simulink library "DCT_Vehicle_Dynamics_Lib"  (R2025a)
settings: Solver=ode45  StartTime=0.0  StopTime=10.0  RelTol=1e-3  EnableMultiTasking=on
undefined symbols (not defined in the file): DCT_Param
libraries: fl_lib x26, nesl_utility x9, sdl_lib x5
Description:
  | Copyright 2014-2025 The MathWorks, Inc.
settings Model: Creator=smiller  LastModifiedBy=smiller
settings SolverCC: AlgebraicLoopSolver=TrustRegion
settings DataIOCC: LimitDataPoints=on  SaveFormat=Array  SignalLoggingSaveFormat=ModelDataLogs  ReturnWorkspaceOutputs=off
settings OptimizationCC: ReuseModelBlockBuffer=off  ExpressionDepthLimit=2147483647.0  LifeSpan=inf
settings DebuggingCC: UnderspecifiedInitializationDetection=Classic  MergeDetectMultiDrivingBlocksExec=none  SolverPrmCheckMsg=warning  FcnCallInpInsideContextMsg=warning  UnconnectedInputMsg=warning  UnconnectedOutputMsg=warning  UnconnectedLineMsg=warning  AllowSymbolicDim=off  StateNameClashWarn=warning  PregeneratedLibrarySubsystemCodeDiagnostic=none  SFUnexpectedBacktrackingDiag=warning  SFNoUnconditionalDefaultTransitionDiag=warning  SFExecutionAtInitializationDiag=none  ArithmeticOperatorsInVariantConditions=warning
settings HardwareCC: ProdBitPerPointer=32.0  ProdBitPerSizeT=32.0  ProdBitPerPtrDiffT=32.0  ProdLargestAtomicFloat=None  ProdIntDivRoundTo=Undefined  ProdEndianess=Unspecified  ProdWordSize=32.0  ProdHWDeviceType=32-bit Generic
settings ModelReferenceCC: EnableRefExpFcnMdlSchedulingChecks=on  PropagateSignalLabelsOutOfModel=off
settings SFSimCC: SimUseLocalCustomCode=off  CustomCodeUndefinedFunction=UseInterfaceOnly
settings RTWCC: RTWUseLocalCustomCode=off  GPUComputeCapability=3.5  DLArmComputeVersion=19.05
settings CodeAppCC: StateflowObjectComments=on
settings GRTTargetCC: TargetLangStandard=C89/C90 (ANSI)  CombineOutputUpdateFcns=off  GRTInterface=on
settings ConfigComp: CovMetricSettings=dw  CovSaveCumulativeToWorkspaceVar=on  CovSaveSingleToWorkspaceVar=on  CovExternalEMLEnable=off  CovSFcnEnable=off

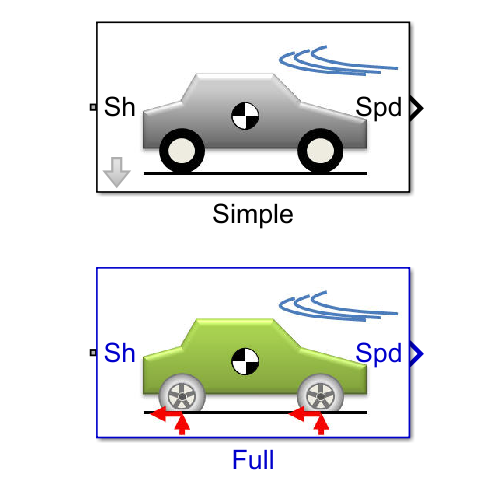
[thumbnail: Simulink's stored preview of the top-level diagram]
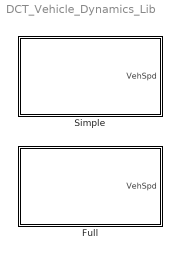
== system DCT_Vehicle_Dynamics_Lib ==
  Full : Subsystem
      mask Display:
      | image(imread('DCT_Vehicle_Dynamics_Full_IMAGE.jpg'));
      | port_label('LConn',1,'Sh');
      | port_label('output',1,'Spd');
  Simple : Subsystem  mask(Rigid vehicle model){mass=DCT_Param.Vehicle.Mass, area=DCT_Param.Vehicle.Frontal_Area, Cd=DCT_Param.Vehicle.Aero_Drag_Coeff, radius=DCT_Param.Vehicle.Tire.Radius, wheel_inertia=DCT_Param.Vehicle.Tire.Inertia, gear_ratio=DCT_Param.Vehicle.Final_Drive_Ratio}
      mask prompts: mass "Vehicle mass (Kg)"; area "Vehicle Area (m^2)"; Cd "Aerodynamic drag coefficient (unitless)"; radius "Tire radius (m)"; wheel_inertia "Total wheel inertia (kg*m^2)"; gear_ratio "Engine to vehicle gear ratio"
      mask help: Model vehicle effective inertia and drag force as seen by the engine. It is assumed that the vehicle is moving on flat terrain. No bearing friction or gear losses are included.
      mask init:
      | gravity = 9.81;
      mask Display:
      | image(imread('DCT_Vehicle_Dynamics_Simple_IMAGE.jpg'));
      | port_label('LConn',1,'Sh');
      | port_label('output',1,'Spd');

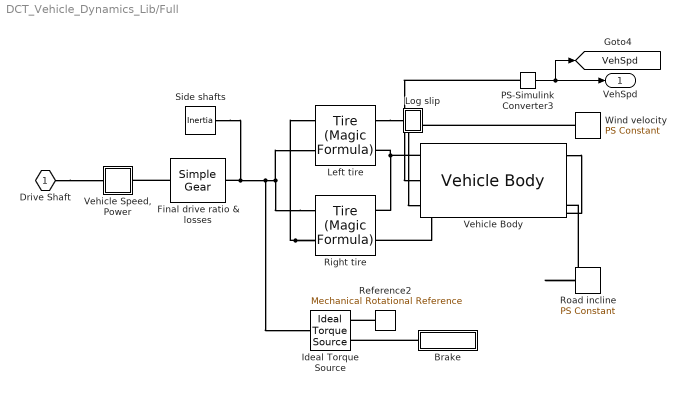
== system DCT_Vehicle_Dynamics_Lib/Full ==
  Brake : Subsystem
  Final drive ratio & losses : sdl_lib/Gears/Simple Gear  ratio=DCT_Param.Vehicle.Final_Drive_Ratio  rotation_direction=3-2*(2)  friction_model=1  T_noload=0.1 N*m  T_nom=5 N*m  efficiency_nom=0.8  efficiency=DCT_Param.Vehicle.Final_Drive_Efficiency  temperature_TLU=[ 280 300 320 ] K  load_TLU=[ 1 5 10 ] N*m  efficiency_TLU=[ 0.95 0.9 0.85 ]  efficiency_TLU2=[ 0.85 0.8 0.75; 0.95 0.9 0.85; 0.85 0.8 0.7 ]  w_thr=DCT_Param.Vehicle.Final_Drive_Vel_Thresh rad/s  pwr_thr=0.001 W  enable_backlash=false  hardstop_model=simscape.enum.hardstop.smooth  backlash_distance=1e-3 mm  r_base=0.1 m  transition=1e-4 mm  backlash_stiffness=1e7 N/m  backlash_damping=1e6 N*s/m  coeff_rest=0  v_tol=0.001 m/s  f_tol=0 N  mu_visc=[0 0] N*m/(rad/s)  thermal_mass=50 J/K  temperature_specify=off  temperature_priority=High  temperature=300 K  temperature_nominal_specify=off  temperature_nominal_value=1  temperature_nominal_unit=K  x_backlash_specify=off  x_backlash_priority=None  x_backlash=0 mm  x_backlash_nominal_specify=off  x_backlash_nominal_value=1  x_backlash_nominal_unit=mm  f_hardstop_specify=off  f_hardstop_priority=None  f_hardstop=0 N  f_hardstop_nominal_specify=off  f_hardstop_nominal_value=1  f_hardstop_nominal_unit=N  v_backlash_specify=off  v_backlash_priority=None  v_backlash=0 m/s  v_backlash_nominal_specify=off  v_backlash_nominal_value=1  v_backlash_nominal_unit=m/s
  Ideal Torque Source : fl_lib/Mechanical/Mechanical Sources/Ideal Torque Source
  Left tire : sdl_lib/Tires & Vehicles/Tire (Magic Formula)  parameterization=3  F_z1=3000 N  F_x1=3500 N  kappa1=10  B_m=10  C_m=1.9  D_m=1  E_m=0.97  fz0=DCT_Param.Vehicle.Tire.Nominal_Vertical_Load N  p_Cx=DCT_Param.Vehicle.Tire.C_Coeff  p_Dx=DCT_Param.Vehicle.Tire.D_Coeff  p_Ex=DCT_Param.Vehicle.Tire.E_Coeff  p_Kx=DCT_Param.Vehicle.Tire.BCD_Coeff  p_Hx=DCT_Param.Vehicle.Tire.H_Coeff  p_Vx=DCT_Param.Vehicle.Tire.V_Coeff  rolling_radius_model=sdl.enum.RollingRadiusParameterization.Constant  r_e=DCT_Param.Vehicle.Tire.Radius m  r_0=0.3 m  breff=8.39  dreff=0.26  freff=0.074  q_re0=0.99  q_v1=0.008  longvl=17 m/s  cz=5e5 N/m  model_resistance=0  resistance_model=1  coeff=0.015  p_tire=250e3 Pa  alpha=-0.003  beta=0.97  coeff_a=84e-4  coeff_b=6.2e-4 s/m  coeff_c=1.6e-4 s^2/m^2  p_tire0=240e3 Pa  fz0_resistance=4000 N  vH0=16 m/s  q_Sy=[.0082, 0, .0014, .001, 0, 0, 1.08, -.5]  v_thr=1e-3 m/s  enable_scaling_coefficients=false  lfzO=1  lcx=1  lmux=1  lex=1  lkx=1  lhx=1  lvx=1  lmy=1  model_compliance=0  stiffness=1e+6 N/m  damping=1000 N/(m/s)  model_inertia=1  inertia=DCT_Param.Vehicle.Tire.Inertia kg*m^2  initial_velocity=DCT_Param.Vehicle.Tire.Initial_Velocity rpm  vxlow=DCT_Param.Vehicle.Tire.Slip_Vel_Thresh m/s  v_tr_thr=0.1*(DCT_Param.Vehicle.Tire.Slip_Vel_Thresh) m/s  kpumin=-1e5  kpumax=1e5
  Log slip : Subsystem
  PS-Simulink Converter3 : nesl_utility/PS-Simulink Converter  PhysicalDomain=network_engine_domain  SubClassName=ps_output  LeftPortType=input  RightPortType=output  PseudoPeriodic=off  Frequencies=[]  VectorFormat=1-D array  Unit=km/hr  AffineConversion=off
  Reference2 : fl_lib/Mechanical/Rotational Elements/Mechanical Rotational Reference
  Right tire : sdl_lib/Tires & Vehicles/Tire (Magic Formula)  parameterization=3  F_z1=3000 N  F_x1=3500 N  kappa1=10  B_m=10  C_m=1.9  D_m=1  E_m=0.97  fz0=DCT_Param.Vehicle.Tire.Nominal_Vertical_Load N  p_Cx=DCT_Param.Vehicle.Tire.C_Coeff  p_Dx=DCT_Param.Vehicle.Tire.D_Coeff  p_Ex=DCT_Param.Vehicle.Tire.E_Coeff  p_Kx=DCT_Param.Vehicle.Tire.BCD_Coeff  p_Hx=DCT_Param.Vehicle.Tire.H_Coeff  p_Vx=DCT_Param.Vehicle.Tire.V_Coeff  rolling_radius_model=sdl.enum.RollingRadiusParameterization.Constant  r_e=DCT_Param.Vehicle.Tire.Radius m  r_0=0.3 m  breff=8.39  dreff=0.26  freff=0.074  q_re0=0.99  q_v1=0.008  longvl=17 m/s  cz=5e5 N/m  model_resistance=0  resistance_model=1  coeff=0.015  p_tire=250e3 Pa  alpha=-0.003  beta=0.97  coeff_a=84e-4  coeff_b=6.2e-4 s/m  coeff_c=1.6e-4 s^2/m^2  p_tire0=240e3 Pa  fz0_resistance=4000 N  vH0=16 m/s  q_Sy=[.0082, 0, .0014, .001, 0, 0, 1.08, -.5]  v_thr=1e-3 m/s  enable_scaling_coefficients=false  lfzO=1  lcx=1  lmux=1  lex=1  lkx=1  lhx=1  lvx=1  lmy=1  model_compliance=0  stiffness=1e+6 N/m  damping=1000 N/(m/s)  model_inertia=1  inertia=DCT_Param.Vehicle.Tire.Inertia kg*m^2  initial_velocity=DCT_Param.Vehicle.Tire.Initial_Velocity rpm  vxlow=DCT_Param.Vehicle.Tire.Slip_Vel_Thresh m/s  v_tr_thr=0.1*(DCT_Param.Vehicle.Tire.Slip_Vel_Thresh) m/s  kpumin=-1e5  kpumax=1e5
  Road incline : fl_lib/Physical Signals/Sources/PS Constant  constant=0
  Side shafts : fl_lib/Mechanical/Rotational Elements/Inertia  inertia=DCT_Param.Vehicle.Side_Shaft_Inertia kg*m^2  num_ports=foundation.enum.numPorts2.one  w_specify=on  w_priority=High  w=DCT_Param.Vehicle.Side_Shaft_Initial_Velocity rad/s  w_nominal_specify=off  w_nominal_value=1  w_nominal_unit=rad/s  t_specify=off  t_priority=High  t=0 N*m  t_nominal_specify=off  t_nominal_value=1  t_nominal_unit=N*m
  Vehicle Body : sdl_lib/Tires & Vehicles/Vehicle Body  mass=DCT_Param.Vehicle.Mass kg  n_w=DCT_Param.Vehicle.Wheels_Per_Axle  x_f=DCT_Param.Vehicle.Distance_CG_FrontAxle m  x_r=DCT_Param.Vehicle.Distance_CG_RearAxle m  y_c=DCT_Param.Vehicle.Distance_CG_Ground m  mass_var=simscape.enum.onoff.off  g=9.81 m/s^2  liftoff_warning=simscape.enum.onoff.off  area=DCT_Param.Vehicle.Frontal_Area m^2  Cd_var=false  Cd=DCT_Param.Vehicle.Aero_Drag_Coeff  rho=1.18 kg/m^3  model_pitch=simscape.enum.onoff.off  inertia=4000 kg*m^2  suspension_model=sdl.enum.linearTLU.linear  k_f=1e4 N/m  b_f=1e4 N/(m/s)  k_r=1e4 N/m  b_r=1e4 N/(m/s)  k_f_TLU=[-2000, -1000, 0, 1000, 2000] N  x_f_TLU=[-.4, -.2, 0, .2, .4] m  b_f_TLU=[-200, -100, 0, 100, 200] N  v_f_TLU=[-4, -2, 0, 2, 4] m/s  k_r_TLU=[-2000, -1000, 0, 1000, 2000] N  x_r_TLU=[-.4, -.2, 0, .2, .4] m  b_r_TLU=[-200, -100, 0, 100, 200] N  v_r_TLU=[-4, -2, 0, 2, 4] m/s  interp_method=simscape.enum.interpolation.linear  extrap_method=simscape.enum.extrapolation.linear  model_hardstop=simscape.enum.onoff.off  upper_bound_f=.25 m  lower_bound_f=-.25 m  stop_k_f=1e6 N/m  stop_b_f=150 N/(m/s)  upper_bound_r=.25 m  lower_bound_r=-.25 m  stop_k_r=1e6 N/m  stop_b_r=150 N/(m/s)  initial_pitch=0 rad  initial_pitch_rate=0 rad/s  v_specify=on  v_priority=High  v=DCT_Param.Vehicle.Initial_Velocity m/s  v_nominal_specify=off  v_nominal_value=1  v_nominal_unit=m/s
      settings: InternalSimscapePortConfiguration="{\"Bottom\":[{\"id\":\"NR\",\"label\":\"NR\",\"type\":\"output\"},{\"id\":\"NF\",\"label\":\"NF\",\"type\":\"output\"},{\"id\":\"beta\",\"label\":\"beta\",\"type\":\"input\"}],\"Left\":[{\"id\":\"H\",\"label\":\"H\",\"type\":\"foundation.mechanical.translational.translational\"}],\"Right\":[],\"Top\":[{\"id\":\"V\",\"label\":\"V\",\"type\":\"output\"},{\"id\":\"wind\",\"label\":\"W\",\"type\":\"input\"}]}"
  "Vehicle Speed, Power" : Subsystem
      mask Display: disp('S')
  Wind velocity : fl_lib/Physical Signals/Sources/PS Constant  constant=0
  Drive Shaft : PMIOPort  Side=Left
  VehSpd : Outport  VectorParamsAs1DForOutWhenUnconnected=off
  tag scope: VehSpd=global
  wires:
  PS-Simulink Converter3/1 -> VehSpd/1, [VehSpd]
  connections:
  Vehicle Body/LConn1 -- Right tire/RConn2 -- Left tire/RConn2
  Right tire/LConn1 -- Left tire/LConn1 -- Vehicle Body/RConn1
  Road incline/RConn1 -- Vehicle Body/RConn3
  Wind velocity/RConn1 -- Vehicle Body/LConn3
  PS-Simulink Converter3/LConn1 -- Vehicle Body/LConn2
  Left tire/RConn1 -- Log slip/LConn1
  Drive Shaft/RConn1 -- "Vehicle Speed, Power"/LConn1
  Brake/RConn1 -- Ideal Torque Source/RConn1
  Reference2/LConn1 -- Ideal Torque Source/RConn2
  Final drive ratio & losses/LConn1 -- "Vehicle Speed, Power"/RConn1
  Right tire/LConn2 -- Left tire/LConn2 -- Final drive ratio & losses/RConn1 -- Side shafts/LConn1 -- Ideal Torque Source/LConn1

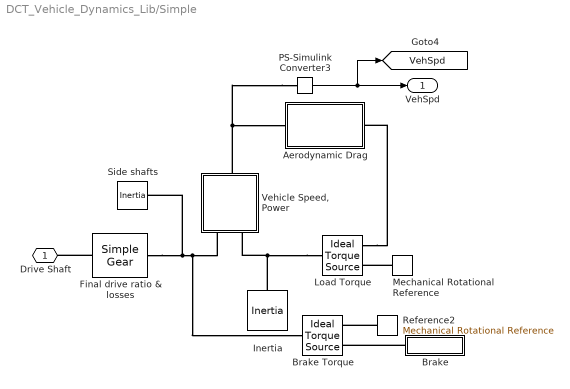
== system DCT_Vehicle_Dynamics_Lib/Simple ==
  Aerodynamic Drag : Subsystem
  Brake : Subsystem
  Brake Torque : fl_lib/Mechanical/Mechanical Sources/Ideal Torque Source
  Final drive ratio & losses : sdl_lib/Gears/Simple Gear  ratio=gear_ratio  rotation_direction=3-2*(2)  friction_model=1  T_noload=0.1 N*m  T_nom=5 N*m  efficiency_nom=0.8  efficiency=DCT_Param.Vehicle.Final_Drive_Efficiency  temperature_TLU=[ 280 300 320 ] K  load_TLU=[ 1 5 10 ] N*m  efficiency_TLU=[ 0.95 0.9 0.85 ]  efficiency_TLU2=[ 0.85 0.8 0.75; 0.95 0.9 0.85; 0.85 0.8 0.7 ]  w_thr=DCT_Param.Vehicle.Final_Drive_Vel_Thresh rad/s  pwr_thr=0.001 W  enable_backlash=false  hardstop_model=simscape.enum.hardstop.smooth  backlash_distance=1e-3 mm  r_base=0.1 m  transition=1e-4 mm  backlash_stiffness=1e7 N/m  backlash_damping=1e6 N*s/m  coeff_rest=0  v_tol=0.001 m/s  f_tol=0 N  mu_visc=[0 0] N*m/(rad/s)  thermal_mass=50 J/K  temperature_specify=off  temperature_priority=High  temperature=300 K  temperature_nominal_specify=off  temperature_nominal_value=1  temperature_nominal_unit=K  x_backlash_specify=off  x_backlash_priority=None  x_backlash=0 mm  x_backlash_nominal_specify=off  x_backlash_nominal_value=1  x_backlash_nominal_unit=mm  f_hardstop_specify=off  f_hardstop_priority=None  f_hardstop=0 N  f_hardstop_nominal_specify=off  f_hardstop_nominal_value=1  f_hardstop_nominal_unit=N  v_backlash_specify=off  v_backlash_priority=None  v_backlash=0 m/s  v_backlash_nominal_specify=off  v_backlash_nominal_value=1  v_backlash_nominal_unit=m/s
  Inertia : fl_lib/Mechanical/Rotational Elements/Inertia  inertia=mass*radius*radius kg*m^2  num_ports=foundation.enum.numPorts2.one  w_specify=on  w_priority=High  w=0 rad/s  w_nominal_specify=off  w_nominal_value=1  w_nominal_unit=rad/s  t_specify=off  t_priority=High  t=0 N*m  t_nominal_specify=off  t_nominal_value=1  t_nominal_unit=N*m
  Load Torque : fl_lib/Mechanical/Mechanical Sources/Ideal Torque Source
  Mechanical Rotational Reference : fl_lib/Mechanical/Rotational Elements/Mechanical Rotational Reference
  PS-Simulink Converter3 : nesl_utility/PS-Simulink Converter  PhysicalDomain=network_engine_domain  SubClassName=ps_output  LeftPortType=input  RightPortType=output  PseudoPeriodic=off  Frequencies=[]  VectorFormat=1-D array  Unit=km/hr  AffineConversion=off
  Reference2 : fl_lib/Mechanical/Rotational Elements/Mechanical Rotational Reference
  Side shafts : fl_lib/Mechanical/Rotational Elements/Inertia  inertia=DCT_Param.Vehicle.Side_Shaft_Inertia+2*wheel_inertia kg*m^2  num_ports=foundation.enum.numPorts2.one  w_specify=on  w_priority=High  w=DCT_Param.Vehicle.Side_Shaft_Initial_Velocity rad/s  w_nominal_specify=off  w_nominal_value=1  w_nominal_unit=rad/s  t_specify=off  t_priority=High  t=0 N*m  t_nominal_specify=off  t_nominal_value=1  t_nominal_unit=N*m
  "Vehicle Speed, Power" : Subsystem
  Drive Shaft : PMIOPort  Side=Left
  VehSpd : Outport  VectorParamsAs1DForOutWhenUnconnected=off
  tag scope: VehSpd=global
  wires:
  PS-Simulink Converter3/1 -> VehSpd/1, [VehSpd]
  connections:
  Final drive ratio & losses/LConn1 -- Drive Shaft/RConn1
  PS-Simulink Converter3/LConn1 -- "Vehicle Speed, Power"/RConn1 -- Aerodynamic Drag/LConn1
  Load Torque/RConn1 -- Aerodynamic Drag/RConn1
  Mechanical Rotational Reference/LConn1 -- Load Torque/RConn2
  Load Torque/LConn1 -- Inertia/LConn1 -- "Vehicle Speed, Power"/LConn2
  Final drive ratio & losses/RConn1 -- "Vehicle Speed, Power"/LConn1 -- Brake Torque/LConn1 -- Side shafts/LConn1
  Brake/RConn1 -- Brake Torque/RConn1
  Reference2/LConn1 -- Brake Torque/RConn2

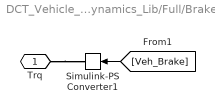
== system DCT_Vehicle_Dynamics_Lib/Full/Brake ==
  Simulink-PS Converter1 : nesl_utility/Simulink-PS Converter  PhysicalDomain=network_engine_domain  SubClassName=ps_input  LeftPortType=input  RightPortType=output  PseudoPeriodic=off  Frequencies=[]  NoiseDistribution=none  NoiseParameters=[]  Unit=1  AffineConversion=off  FilteringAndDerivatives=zero  SimscapeFilterOrder=1  InputFilterTimeConstant=0.005  UdotUserProvided=0
  Trq : PMIOPort  Side=Right
  wires:
  [Veh_Brake] -> Simulink-PS Converter1/1
  connections:
  Trq/RConn1 -- Simulink-PS Converter1/RConn1

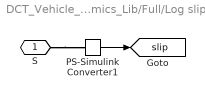
== system DCT_Vehicle_Dynamics_Lib/Full/Log slip ==
  PS-Simulink Converter1 : nesl_utility/PS-Simulink Converter  PhysicalDomain=network_engine_domain  SubClassName=ps_output  LeftPortType=input  RightPortType=output  PseudoPeriodic=off  Frequencies=[]  VectorFormat=1-D array  Unit=1  AffineConversion=off
  S : PMIOPort  Side=Left
  tag scope: slip=global
  wires:
  PS-Simulink Converter1/1 -> [slip]
  connections:
  S/RConn1 -- PS-Simulink Converter1/LConn1

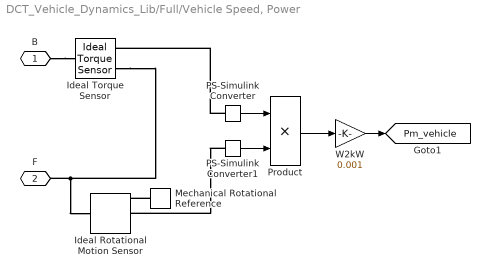
== system DCT_Vehicle_Dynamics_Lib/Full/Vehicle Speed, Power ==
  Ideal Rotational Motion Sensor : fl_lib/Mechanical/Mechanical Sensors/Ideal Rotational Motion Sensor  reference=foundation.enum.MeasurementReference.difference  acceleration_port=false  velocity_port=true  position_port=true  wrap_angle=simscape.enum.onoff.off  offset=0 rad
  Ideal Torque Sensor : fl_lib/Mechanical/Mechanical Sensors/Ideal Torque Sensor
  Mechanical Rotational Reference : fl_lib/Mechanical/Rotational Elements/Mechanical Rotational Reference
  PS-Simulink Converter : nesl_utility/PS-Simulink Converter  PhysicalDomain=network_engine_domain  SubClassName=ps_output  LeftPortType=input  RightPortType=output  PseudoPeriodic=off  Frequencies=[]  VectorFormat=1-D array  Unit=N*m  AffineConversion=off
  PS-Simulink Converter1 : nesl_utility/PS-Simulink Converter  PhysicalDomain=network_engine_domain  SubClassName=ps_output  LeftPortType=input  RightPortType=output  PseudoPeriodic=off  Frequencies=[]  VectorFormat=1-D array  Unit=rad/s  AffineConversion=off
  Product : Product  RndMeth=Zero
  W2kW : Gain  Gain=0.001
  B : PMIOPort  Side=Left
  F : PMIOPort  Port=2  Side=Right
  tag scope: Pm_vehicle=global
  wires:
  PS-Simulink Converter1/1 -> Product/2
  PS-Simulink Converter/1 -> Product/1
  Product/1 -> W2kW/1
  W2kW/1 -> [Pm_vehicle]
  connections:
  PS-Simulink Converter1/LConn1 -- Ideal Rotational Motion Sensor/RConn2
  PS-Simulink Converter/LConn1 -- Ideal Torque Sensor/RConn2
  B/RConn1 -- Ideal Torque Sensor/LConn1
  Ideal Torque Sensor/RConn1 -- F/RConn1 -- Ideal Rotational Motion Sensor/LConn1
  Mechanical Rotational Reference/LConn1 -- Ideal Rotational Motion Sensor/RConn1

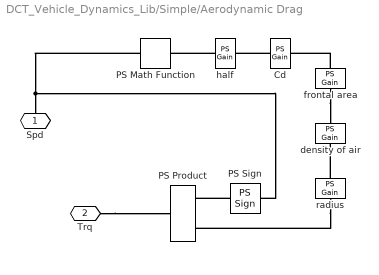
== system DCT_Vehicle_Dynamics_Lib/Simple/Aerodynamic Drag ==
  Cd : fl_lib/Physical Signals/Functions/PS Gain  gain=Cd
  PS Math Function : fl_lib/Physical Signals/Functions/PS Math Function  fcn_choice=7  v=1
  PS Product : fl_lib/Physical Signals/Functions/PS Product
  PS Sign : fl_lib/Physical Signals/Nonlinear Operators/PS Sign
      settings: InternalSimscapePortConfiguration="{\"Bottom\":[],\"Left\":[{\"id\":\"I\",\"label\":\"\",\"type\":\"input\"}],\"Right\":[{\"id\":\"O\",\"label\":\"\",\"type\":\"output\"}],\"Top\":[]}"
  density of air : fl_lib/Physical Signals/Functions/PS Gain  gain=1.2 kg/m^3
  frontal area : fl_lib/Physical Signals/Functions/PS Gain  gain=area m^2
  half : fl_lib/Physical Signals/Functions/PS Gain  gain=1/2
  radius : fl_lib/Physical Signals/Functions/PS Gain  gain=-radius m
  Spd : PMIOPort  Side=Left
  Trq : PMIOPort  Port=2  Side=Right
  connections:
  frontal area/RConn1 -- density of air/LConn1
  frontal area/LConn1 -- Cd/RConn1
  radius/LConn1 -- density of air/RConn1
  PS Sign/RConn1 -- PS Product/LConn2
  radius/RConn1 -- PS Product/LConn1
  Cd/LConn1 -- half/RConn1
  half/LConn1 -- PS Math Function/RConn1
  PS Math Function/LConn1 -- PS Sign/LConn1 -- Spd/RConn1
  Trq/RConn1 -- PS Product/RConn1

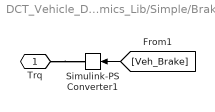
== system DCT_Vehicle_Dynamics_Lib/Simple/Brake ==
  Simulink-PS Converter1 : nesl_utility/Simulink-PS Converter  PhysicalDomain=network_engine_domain  SubClassName=ps_input  LeftPortType=input  RightPortType=output  PseudoPeriodic=off  Frequencies=[]  NoiseDistribution=none  NoiseParameters=[]  Unit=1  AffineConversion=off  FilteringAndDerivatives=zero  SimscapeFilterOrder=1  InputFilterTimeConstant=0.005  UdotUserProvided=0
  Trq : PMIOPort  Side=Right
  wires:
  [Veh_Brake] -> Simulink-PS Converter1/1
  connections:
  Trq/RConn1 -- Simulink-PS Converter1/RConn1

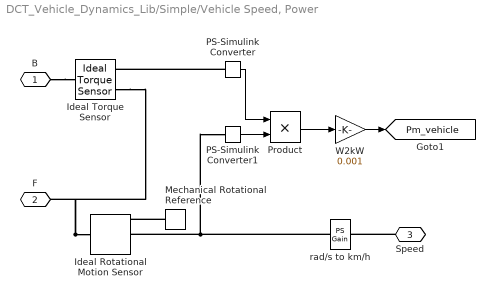
== system DCT_Vehicle_Dynamics_Lib/Simple/Vehicle Speed, Power ==
  Ideal Rotational Motion Sensor : fl_lib/Mechanical/Mechanical Sensors/Ideal Rotational Motion Sensor  reference=foundation.enum.MeasurementReference.difference  acceleration_port=false  velocity_port=true  position_port=true  wrap_angle=simscape.enum.onoff.off  offset=0 rad
  Ideal Torque Sensor : fl_lib/Mechanical/Mechanical Sensors/Ideal Torque Sensor
  Mechanical Rotational Reference : fl_lib/Mechanical/Rotational Elements/Mechanical Rotational Reference
  PS-Simulink Converter : nesl_utility/PS-Simulink Converter  PhysicalDomain=network_engine_domain  SubClassName=ps_output  LeftPortType=input  RightPortType=output  PseudoPeriodic=off  Frequencies=[]  VectorFormat=1-D array  Unit=N*m  AffineConversion=off
  PS-Simulink Converter1 : nesl_utility/PS-Simulink Converter  PhysicalDomain=network_engine_domain  SubClassName=ps_output  LeftPortType=input  RightPortType=output  PseudoPeriodic=off  Frequencies=[]  VectorFormat=1-D array  Unit=rad/s  AffineConversion=off
  Product : Product  RndMeth=Zero
  W2kW : Gain  Gain=0.001
  rad/s to km/h : fl_lib/Physical Signals/Functions/PS Gain  gain=radius*3.6 (km/hr)/(rad/s)
  B : PMIOPort  Side=Left
  F : PMIOPort  Port=2  Side=Left
  Speed : PMIOPort  Port=3  Side=Right
  tag scope: Pm_vehicle=global
  wires:
  W2kW/1 -> [Pm_vehicle]
  Product/1 -> W2kW/1
  PS-Simulink Converter/1 -> Product/1
  PS-Simulink Converter1/1 -> Product/2
  connections:
  Mechanical Rotational Reference/LConn1 -- Ideal Rotational Motion Sensor/RConn1
  Ideal Rotational Motion Sensor/LConn1 -- F/RConn1 -- Ideal Torque Sensor/RConn1
  B/RConn1 -- Ideal Torque Sensor/LConn1
  PS-Simulink Converter/LConn1 -- Ideal Torque Sensor/RConn2
  rad/s to km/h/LConn1 -- Ideal Rotational Motion Sensor/RConn2 -- PS-Simulink Converter1/LConn1
  Speed/RConn1 -- rad/s to km/h/RConn1
